simulink model "FSI03"  (R2024b)
settings: Solver=VariableStepAuto  StartTime=0.0  StopTime=1  RelTol=1e-3
values from neighbouring files (symbols this model uses):
  b = 350    [FSI03WS.m]    (also in FSI04WS.m = 5; FSI08WS.m = 1.25663706144; FSI09WS.m = 3.14159265359)
  C = 0.01    [FSI03WS.m]    (also in FSI09WS.m = [1 0])
  g = 10    [FSI03WS.m]
  I0 = 0    [FSI03WS.m]    (also in FSI05WS.m = 0.0001; FSI06WS.m = 0.0001; FSI07WS.m = 0.0001)
  L = 0.02    [FSI03WS.m]    (also in FSI05WS.m = 0.05; FSI06WS.m = 0.05; FSI07WS.m = 0.05; FSI10WS.m = 0.3)
  m = 70    [FSI03WS.m]    (also in FSI04WS.m = 2; FSI08WS.m = 1; FSI09WS.m = 4; FSI10WS.m = 2)
  R = 5    [FSI03WS.m]    (also in FSI05WS.m = 0; FSI06WS.m = 20; FSI07WS.m = 20)
  U = 10    [FSI03WS.m]    (also in FSI05WS.m = 24; FSI06WS.m = 24)
  v_0 = 0    [FSI03WS.m]
settings Model: Creator=fmiro  LastModifiedBy=fmiro

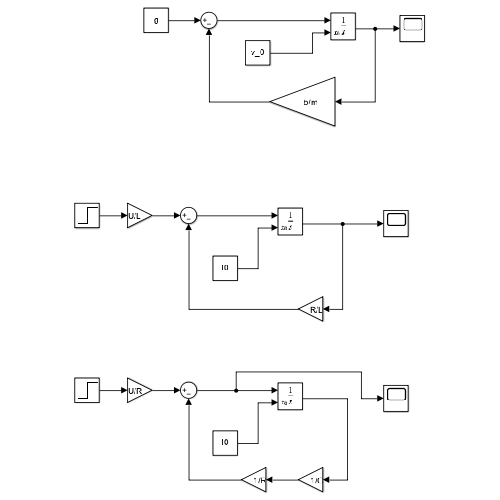
[thumbnail: Simulink's stored preview of the top-level diagram]
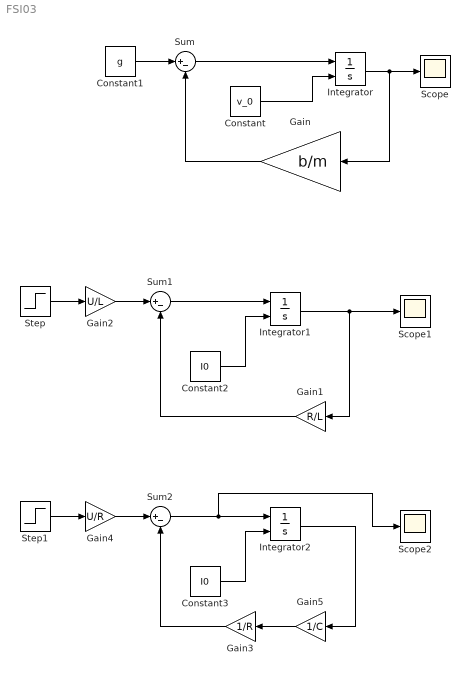
== system FSI03 ==
  Constant : Constant  Value=v_0
  Constant1 : Constant  Value=g
  Constant2 : Constant  Value=I0
  Constant3 : Constant  Value=I0
  Gain : Gain  Gain=b/m
  Gain1 : Gain  Gain=R/L
  Gain2 : Gain  Gain=U/L
  Gain3 : Gain  Gain=1/R
  Gain4 : Gain  Gain=U/R
  Gain5 : Gain  Gain=1/C
  Integrator : Integrator  InitialConditionSource=external
  Integrator1 : Integrator  InitialConditionSource=external
  Integrator2 : Integrator  InitialConditionSource=external
  Scope : Scope
  Scope1 : Scope
  Scope2 : Scope
  Step : Step  Time=0.1  SampleTime=0
  Step1 : Step  Time=0.1  SampleTime=0
  Sum : Sum  Inputs=|+-
  Sum1 : Sum  Inputs=|+-
  Sum2 : Sum  Inputs=|+-
  wires:
  Constant1/1 -> Sum/1
  Sum/1 -> Integrator/1
  Integrator/1 -> Scope/1, Gain/1
  Gain/1 -> Sum/2
  Constant/1 -> Integrator/2
  Constant2/1 -> Integrator1/2
  Integrator1/1 -> Gain1/1, Scope1/1
  Gain1/1 -> Sum1/2
  Sum1/1 -> Integrator1/1
  Step/1 -> Gain2/1
  Gain2/1 -> Sum1/1
  Gain4/1 -> Sum2/1
  Step1/1 -> Gain4/1
  Sum2/1 -> Scope2/1, Integrator2/1
  Gain3/1 -> Sum2/2
  Integrator2/1 -> Gain5/1
  Constant3/1 -> Integrator2/2
  Gain5/1 -> Gain3/1
